simulink model "HW7"  (R2023b)
settings: Solver=VariableStepAuto  StartTime=0.0  StopTime=100  RelTol=1e-3
InitFcn:
  | clear
  | s=tf('s');
  | G=1/(s+1)^3;
  | Ti=1;
  | K=0.15;
  | PI_C=K*(1+1/(Ti*s))
libraries: cstblocks x4
settings Model: Creator=061  LastModifiedBy=ArshiaGosh
settings DebuggingCC: UnconnectedInputMsg=warning  UnconnectedOutputMsg=warning  UnconnectedLineMsg=warning
settings ModelReferenceCC: EnableRefExpFcnMdlSchedulingChecks=on
settings RTWCC: DLArmComputeVersion=19.05

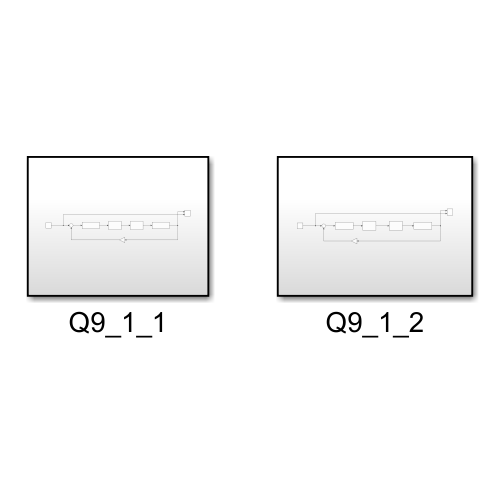
[thumbnail: Simulink's stored preview of the top-level diagram]
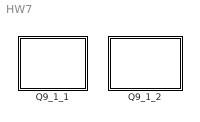
== system HW7 ==
  Q9_1_1 : Subsystem
  Q9_1_2 : Subsystem

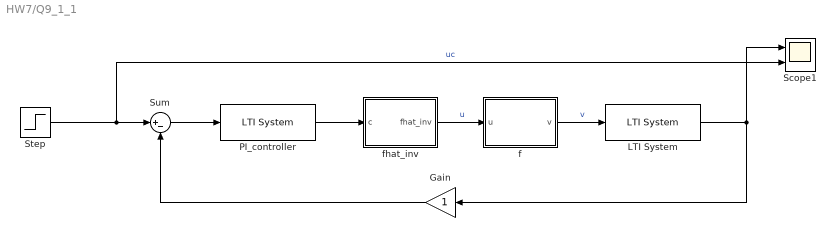
== system HW7/Q9_1_1 ==
  Gain : Gain
  LTI System : cstblocks/LTI System  sys=G  IC=[]  PadeOrder=0
  PI_controller : cstblocks/LTI System  sys=PI_C  IC=[]  PadeOrder=0
  Scope1 : Scope  NumInputPorts=2
  Step : Step  Time=0  After=1.1  SampleTime=0
  Sum : Sum  Inputs=|+-
  f : MATLAB Function  TreatAsAtomicUnit=on
  fhat_inv : MATLAB Function  TreatAsAtomicUnit=on
  wires:
  fhat_inv/1(fhat_inv) -> f/1(u)  "u"
  LTI System/1 -> Scope1/1, Gain/1
  PI_controller/1 -> fhat_inv/1(c)
  Step/1 -> Scope1/2, Sum/1  "uc"
  Gain/1 -> Sum/2
  Sum/1 -> PI_controller/1
  f/1(v) -> LTI System/1  "v"

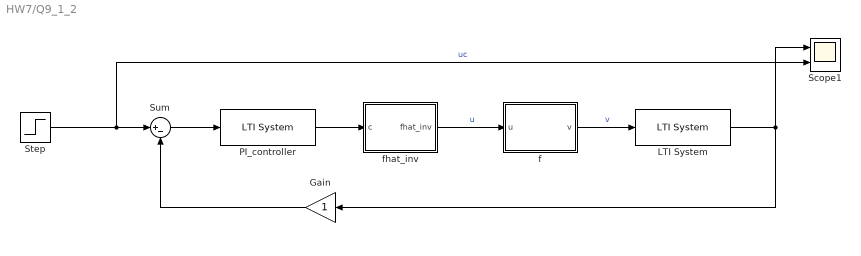
== system HW7/Q9_1_2 ==
  Gain : Gain
  LTI System : cstblocks/LTI System  sys=G  IC=[]  PadeOrder=0
  PI_controller : cstblocks/LTI System  sys=PI_C  IC=[]  PadeOrder=0
  Scope1 : Scope  NumInputPorts=2
  Step : Step  Time=0  After=1.1  SampleTime=0
  Sum : Sum  Inputs=|+-
  f : MATLAB Function  TreatAsAtomicUnit=on
  fhat_inv : MATLAB Function  TreatAsAtomicUnit=on
  wires:
  f/1(v) -> LTI System/1  "v"
  Sum/1 -> PI_controller/1
  Gain/1 -> Sum/2
  Step/1 -> Scope1/2, Sum/1  "uc"
  PI_controller/1 -> fhat_inv/1(c)
  LTI System/1 -> Scope1/1, Gain/1
  fhat_inv/1(fhat_inv) -> f/1(u)  "u"

== matlab function HW7/Q9_1_1/fhat_inv ==
  data: c input; fhat_inv output
function fhat_inv = fcn(c)
if c>=0 && c<=3
fhat_inv=0.433*c;
elseif c>=3 && c<=16
fhat_inv=0.0538*c+1.139;
else
  fhat_inv=0;
end

== matlab function HW7/Q9_1_2/f ==
  data: u input; v output
function v = fcn(u)
v=u^4;

== matlab function HW7/Q9_1_2/fhat_inv ==
  data: c input; fhat_inv output
function fhat_inv = fcn(c)
if c>=0 && c<2
fhat_inv=0.55*c;
elseif c>=2 && c<3.5
fhat_inv=0.2*c+.7;
elseif c>=3.5 && c<5.5
  fhat_inv=0.15*c+0.87;
else
    fhat_inv=0.0286*c+1.5571;
end

== matlab function HW7/Q9_1_1/f ==
  data: u input; v output
function v = fcn(u)
v=u^4;
